simulink model "H2H8"  (R2024a)
settings: Solver=ode15s  StartTime=0.0  StopTime=10.0  FixedStep=0.01  MaxStep=0.01  RelTol=1e-3
values from neighbouring files (symbols this model uses):
  k_h2hinf = H2H8_Regulation(A,B,E,C,D,Dw)    [controlloH2H8_H8alfa.m]
  k_hinfalfa = HinfRstability_regulation(A,B,E,C,Dw,D,70,80,pi/4)    [controlloH2H8_H8alfa.m]
  params = [    690 ... (first row only)    [L1_H2_Hinf_dosso.m]    (also in L1_H2_Hinf_strada_dissestata.m; controlloH2H8_H8alfa.m; controlloH2Robusto.m; controlloH2_dinamico.m)
  x0 = zeros(8,1)    [L1_H2_Hinf_dosso.m]    (also in L1_H2_Hinf_strada_dissestata.m; controlloH2H8_H8alfa.m; controlloH2Robusto.m; controlloH2_dinamico.m)
settings Model: Creator=alest  LastModifiedBy=alest

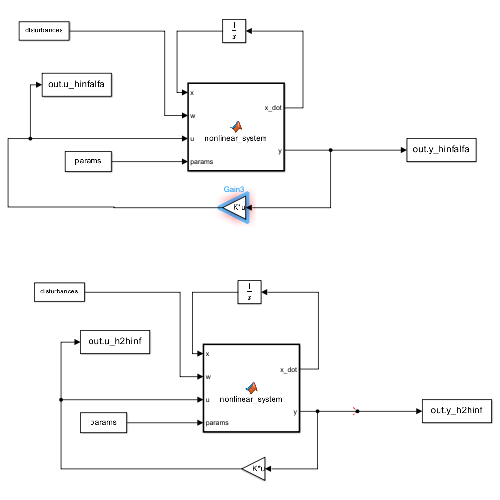
[thumbnail: Simulink's stored preview of the top-level diagram]
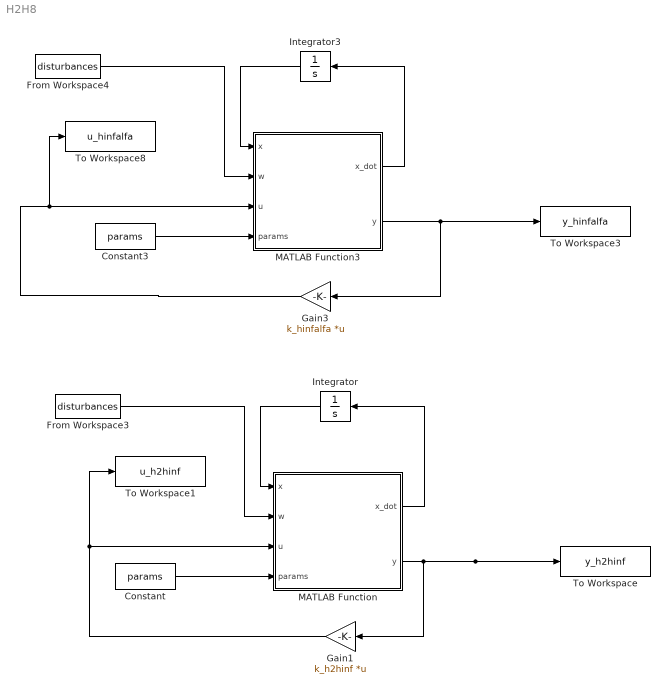
== system H2H8 ==
  Constant : Constant  Value=params
  Constant3 : Constant  Value=params
  From Workspace3 : FromWorkspace  VariableName=disturbances
  From Workspace4 : FromWorkspace  VariableName=disturbances
  Gain1 : Gain  Gain=k_h2hinf  Multiplication=Matrix(K*u)
  Gain3 : Gain  Gain=k_hinfalfa  Multiplication=Matrix(K*u)
  Integrator : Integrator  InitialCondition=x0
  Integrator3 : Integrator  InitialCondition=x0
  MATLAB Function : MATLAB Function  TreatAsAtomicUnit=on
  MATLAB Function3 : MATLAB Function  TreatAsAtomicUnit=on
  To Workspace : ToWorkspace  VariableName=y_h2hinf  SaveFormat=Timeseries  SampleTime=-1
  To Workspace1 : ToWorkspace  VariableName=u_h2hinf  SaveFormat=Timeseries  SampleTime=-1
  To Workspace3 : ToWorkspace  VariableName=y_hinfalfa  SaveFormat=Timeseries  SampleTime=-1
  To Workspace8 : ToWorkspace  VariableName=u_hinfalfa  SaveFormat=Timeseries  SampleTime=-1
  wires:
  Integrator/1 -> MATLAB Function/1(x)
  MATLAB Function/1(x_dot) -> Integrator/1
  MATLAB Function/2(y) -> Gain1/1, To Workspace/1
  From Workspace3/1 -> MATLAB Function/2(w)
  Constant/1 -> MATLAB Function/4(params)
  Gain1/1 -> To Workspace1/1, MATLAB Function/3(u)
  Gain3/1 -> To Workspace8/1, MATLAB Function3/3(u)
  Constant3/1 -> MATLAB Function3/4(params)
  From Workspace4/1 -> MATLAB Function3/2(w)
  Integrator3/1 -> MATLAB Function3/1(x)
  MATLAB Function3/2(y) -> Gain3/1, To Workspace3/1
  MATLAB Function3/1(x_dot) -> Integrator3/1

== matlab function H2H8/MATLAB Function ==
  data: x input; w input; u input; params input; x_dot output; y output
function [x_dot,y] = nonlinear_system(x, w, u, params)
% HALF_CAR_NONLINEAR Modello non lineare di un sistema "half-car" nello spazio di stato.
%
% Input:
%   t      - Tempo (non usato nel calcolo, ma utile per simulazioni)
%   x      - Stato del sistema [x1; x2; x3; x4; x5; x6; x7; x8]
%            x1: z_s    (posizione verticale della massa sospesa)
%            x2: z_s_dot (velocità verticale della massa sospesa)
%            x3: psi    (angolo di beccheggio)
%            x4: psi_dot (velocità angolare di beccheggio)
%            x5: z_uf   (posizione verticale ruota anteriore)
%            x6: z_uf_dot (velocità verticale ruota anteriore)
%            x7: z_ur   (posizione verticale ruota posteriore)
%            x8: z_ur_dot (velocità verticale ruota posteriore)
%   u      - Ingressi [u_f; u_r] (forze applicate alle ruote anteriore e posteriore)
%   z_rf   - Profilo stradale ruota anteriore
%   z_rr   - Profilo stradale ruota posteriore
%   params - Parametri del sistema (struttura con campi):
%            m_s, I_psi, L_f, L_r, k_sf, c_sf, k_sr, c_sr, m_uf, m_ur, k_uf, k_ur
%
% Output:
%   x_dot - Derivate dello stato [x1_dot; x2_dot; ...; x8_dot]

% Estrai parametri
    m_s   = params(1);
    I_psi = params(2);
    L_f   = params(3);
    L_r   = params(4);
    k_sf  = params(5);
    c_sf  = params(6);
    k_sr  = params(7);
    c_sr  = params(8);
    m_uf  = params(9);
    m_ur  = params(10);
    k_uf  = params(11);
    k_ur  = params(12);
% Estrai stati
z_s = x(1);      z_s_dot = x(2);
psi = x(3);      psi_dot = x(4);
z_uf = x(5);     z_uf_dot = x(6);
z_ur = x(7);     z_ur_dot = x(8);

% Estrai disturbi
z_rf = w(1);  % profilo stradale anteriore
z_rr = w(2);  % profilo stradale posteriore

% Estrai ingressi
u_f = u(1);  % Forza ruota anteriore
u_r = u(2);  % Forza ruota posteriore

% Calcola z_sf e z_sr (posizioni cinematiche)
z_sf = z_s - L_f * sin(psi);
z_sr = z_s + L_r * sin(psi);

% Calcola z_sf_dot e z_sr_dot (velocità cinematiche)
z_sf_dot = z_s_dot - L_f * cos(psi) * psi_dot;
z_sr_dot = z_s_dot + L_r * cos(psi) * psi_dot;

% Equazioni del sistema nello spazio di stato
z_s_ddot = (1/m_s) * ( ...
    -k_sf * (z_sf - z_uf) - c_sf * (z_sf_dot - z_uf_dot) ...
    -k_sr * (z_sr - z_ur) - c_sr * (z_sr_dot - z_ur_dot) ...
    + u_f + u_r);

psi_ddot = (1/I_psi) * ( ...
    L_f * cos(psi) * (k_sf * (z_sf - z_uf) + c_sf * (z_sf_dot - z_uf_dot)) ...
    - L_r * cos(psi) * (k_sr * (z_sr - z_ur) + c_sr * (z_sr_dot - z_ur_dot)) ...
    - L_f * cos(psi) * u_f + L_r * cos(psi) * u_r);

z_uf_ddot = (1/m_uf) * ( ...
    -k_uf * (z_uf - z_rf) - k_sf * (z_uf - z_sf) - c_sf * (z_uf_dot - z_sf_dot) ...
    - u_f);

z_ur_ddot = (1/m_ur) * ( ...
    -k_ur * (z_ur - z_rr) - k_sr * (z_ur - z_sr) - c_sr * (z_ur_dot - z_sr_dot) ...
    - u_r);

% Stato derivato
x_dot = [z_s_dot;           % x1_dot
         z_s_ddot;          % x2_dot
         psi_dot;           % x3_dot
         psi_ddot;          % x4_dot
         z_uf_dot;          % x5_dot
         z_uf_ddot;         % x6_dot
         z_ur_dot;          % x7_dot
         z_ur_ddot];        % x8_dot

y=x;

end

== matlab function H2H8/MATLAB Function3 ==
  data: x input; w input; u input; params input; x_dot output; y output
function [x_dot,y] = nonlinear_system(x, w, u, params)
% HALF_CAR_NONLINEAR Modello non lineare di un sistema "half-car" nello spazio di stato.
%
% Input:
%   t      - Tempo (non usato nel calcolo, ma utile per simulazioni)
%   x      - Stato del sistema [x1; x2; x3; x4; x5; x6; x7; x8]
%            x1: z_s    (posizione verticale della massa sospesa)
%            x2: z_s_dot (velocità verticale della massa sospesa)
%            x3: psi    (angolo di beccheggio)
%            x4: psi_dot (velocità angolare di beccheggio)
%            x5: z_uf   (posizione verticale ruota anteriore)
%            x6: z_uf_dot (velocità verticale ruota anteriore)
%            x7: z_ur   (posizione verticale ruota posteriore)
%            x8: z_ur_dot (velocità verticale ruota posteriore)
%   u      - Ingressi [u_f; u_r] (forze applicate alle ruote anteriore e posteriore)
%   z_rf   - Profilo stradale ruota anteriore
%   z_rr   - Profilo stradale ruota posteriore
%   params - Parametri del sistema (struttura con campi):
%            m_s, I_psi, L_f, L_r, k_sf, c_sf, k_sr, c_sr, m_uf, m_ur, k_uf, k_ur
%
% Output:
%   x_dot - Derivate dello stato [x1_dot; x2_dot; ...; x8_dot]

% Estrai parametri
    m_s   = params(1);
    I_psi = params(2);
    L_f   = params(3);
    L_r   = params(4);
    k_sf  = params(5);
    c_sf  = params(6);
    k_sr  = params(7);
    c_sr  = params(8);
    m_uf  = params(9);
    m_ur  = params(10);
    k_uf  = params(11);
    k_ur  = params(12);
% Estrai stati
z_s = x(1);      z_s_dot = x(2);
psi = x(3);      psi_dot = x(4);
z_uf = x(5);     z_uf_dot = x(6);
z_ur = x(7);     z_ur_dot = x(8);

% Estrai disturbi
z_rf = w(1);  % profilo stradale anteriore
z_rr = w(2);  % profilo stradale posteriore

% Estrai ingressi
u_f = u(1);  % Forza ruota anteriore
u_r = u(2);  % Forza ruota posteriore

% Calcola z_sf e z_sr (posizioni cinematiche)
z_sf = z_s - L_f * sin(psi);
z_sr = z_s + L_r * sin(psi);

% Calcola z_sf_dot e z_sr_dot (velocità cinematiche)
z_sf_dot = z_s_dot - L_f * cos(psi) * psi_dot;
z_sr_dot = z_s_dot + L_r * cos(psi) * psi_dot;

% Equazioni del sistema nello spazio di stato
z_s_ddot = (1/m_s) * ( ...
    -k_sf * (z_sf - z_uf) - c_sf * (z_sf_dot - z_uf_dot) ...
    -k_sr * (z_sr - z_ur) - c_sr * (z_sr_dot - z_ur_dot) ...
    + u_f + u_r);

psi_ddot = (1/I_psi) * ( ...
    L_f * cos(psi) * (k_sf * (z_sf - z_uf) + c_sf * (z_sf_dot - z_uf_dot)) ...
    - L_r * cos(psi) * (k_sr * (z_sr - z_ur) + c_sr * (z_sr_dot - z_ur_dot)) ...
    - L_f * cos(psi) * u_f + L_r * cos(psi) * u_r);

z_uf_ddot = (1/m_uf) * ( ...
    -k_uf * (z_uf - z_rf) - k_sf * (z_uf - z_sf) - c_sf * (z_uf_dot - z_sf_dot) ...
    - u_f);

z_ur_ddot = (1/m_ur) * ( ...
    -k_ur * (z_ur - z_rr) - k_sr * (z_ur - z_sr) - c_sr * (z_ur_dot - z_sr_dot) ...
    - u_r);

% Stato derivato
x_dot = [z_s_dot;           % x1_dot
         z_s_ddot;          % x2_dot
         psi_dot;           % x3_dot
         psi_ddot;          % x4_dot
         z_uf_dot;          % x5_dot
         z_uf_ddot;         % x6_dot
         z_ur_dot;          % x7_dot
         z_ur_ddot];        % x8_dot

y=x;
end
